simulink model "hdlcoder_saturate_eml"  (R2026a)
settings: Solver=FixedStepDiscrete  StopTime=1000  FixedStep=1  EnableMultiTasking=on
libraries: simulink x1
settings Model: Creator=The MathWorks, Inc.  LastModifiedBy=The MathWorks, Inc.
settings OptimizationCC: InitFltsAndDblsToZero=on
settings DebuggingCC: UnderspecifiedInitializationDetection=Classic  MultiTaskDSMMsg=warning  MultiTaskCondExecSysMsg=none
settings HardwareCC: ProdHWDeviceType=32-bit Generic
settings GRTTargetCC: CombineOutputUpdateFcns=off  GRTInterface=on

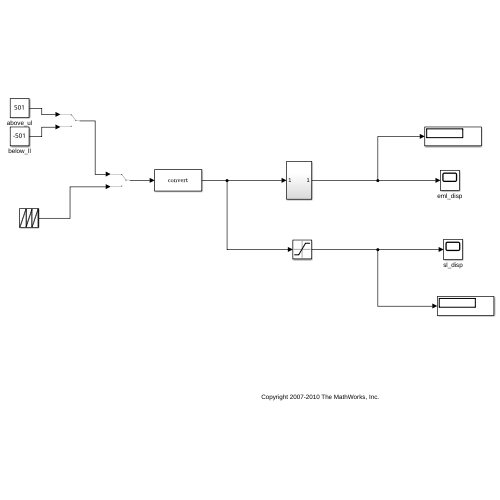
[thumbnail: Simulink's stored preview of the top-level diagram]
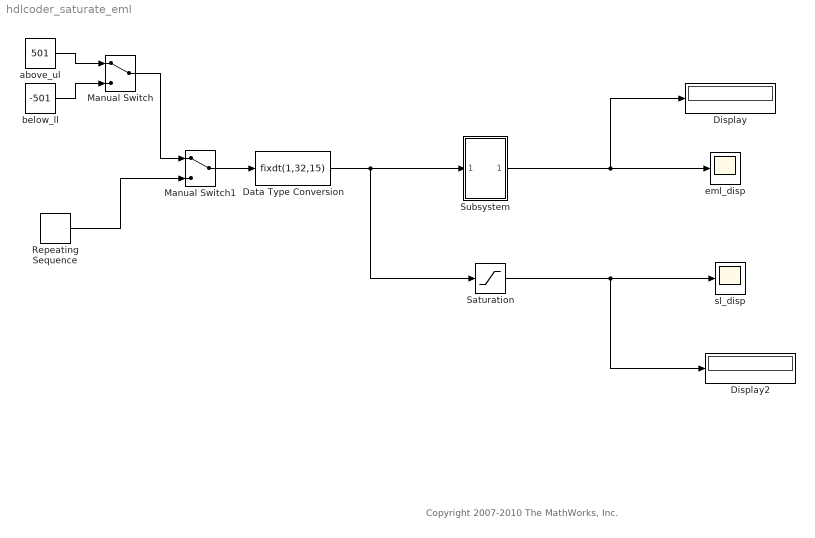
== system hdlcoder_saturate_eml ==
  note: Copyright 2007-2010 The MathWorks, Inc.
  Data Type Conversion : DataTypeConversion  OutDataTypeStr=fixdt(1,32,15)  SaturateOnIntegerOverflow=off  RndMeth=Floor
  Display : Display
  Display2 : Display
  Manual Switch : ManualSwitch
  Manual Switch1 : ManualSwitch
  Repeating Sequence : simulink/Sources/Repeating Sequence  rep_seq_t=[0:110]  rep_seq_y=[-550:10:550]
  Saturation : Saturate  UpperLimit=500  LowerLimit=-500
  Subsystem : Subsystem
  above_ul : Constant  Value=501
  below_ll : Constant  Value=-501
  eml_disp : Scope
  sl_disp : Scope
  wires:
  Data Type Conversion/1 -> Saturation/1, Subsystem/1(In1)
  Saturation/1 -> sl_disp/1, Display2/1
  Subsystem/1(Out1) -> eml_disp/1, Display/1
  above_ul/1 -> Manual Switch/1
  below_ll/1 -> Manual Switch/2
  Manual Switch1/1 -> Data Type Conversion/1
  Manual Switch/1 -> Manual Switch1/1
  Repeating Sequence/1 -> Manual Switch1/2

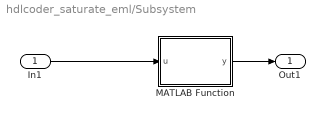
== system hdlcoder_saturate_eml/Subsystem ==
  In1 : Inport
  MATLAB Function : MATLAB Function  TreatAsAtomicUnit=on
  Out1 : Outport
  wires:
  In1/1 -> MATLAB Function/1(u)
  MATLAB Function/1(y) -> Out1/1

== matlab function hdlcoder_saturate_eml/Subsystem/MATLAB Function ==
  data: u input; y output
function y = fcn(u) 
% Implementation of Saturation block.

% Note Input can be integer or fixedpoint type 
% (see this block setting: treat input as int or fi)


upper_limit = fi(500, numerictype(u), fimath(u));
lower_limit = fi(-500, numerictype(u), fimath(u));

if (u > upper_limit)
    y = upper_limit;
elseif (u < lower_limit)
    y = lower_limit;
else
    y = u;
end
